simulink model "prelab10"  (R2021a)
settings: Solver=VariableStepAuto  StartTime=0.0  StopTime=0.005  RelTol=1e-3
settings Model: Creator=Mataya  LastModifiedBy=Mataya

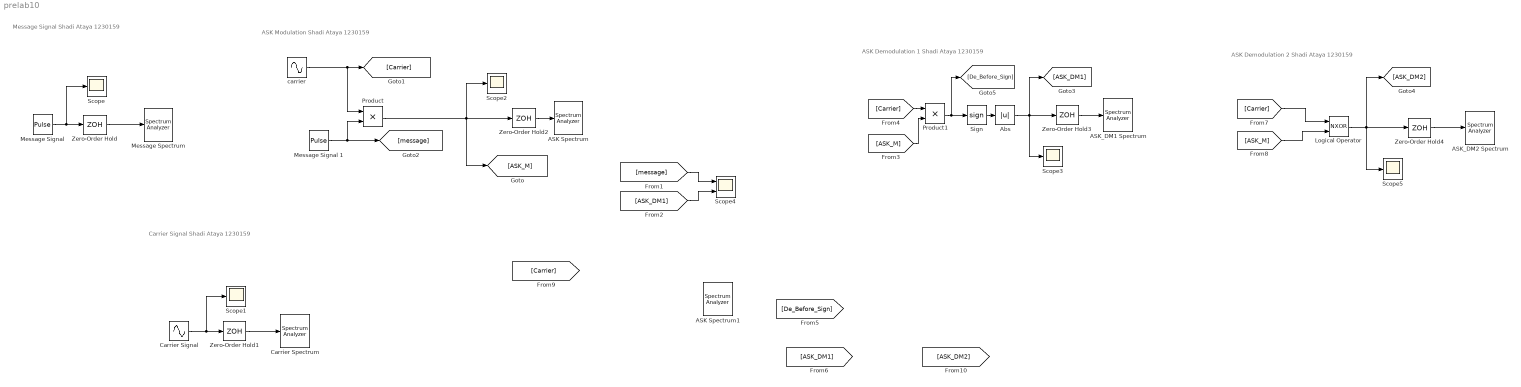
== system prelab10 ==
  note: ASK Demodulation 2
      | Shadi Ataya 1230159
  note: ASK Demodulation 1
      | Shadi Ataya 1230159
  note: ASK Modulation
      | Shadi Ataya 1230159
  note: Message Signal
      | Shadi Ataya 1230159
  note: Carrier Signal
      | Shadi Ataya 1230159
  ASK Spectrum : SpectrumAnalyzer
  ASK Spectrum1 : SpectrumAnalyzer
  ASK_DM1 Spectrum : SpectrumAnalyzer
  ASK_DM2 Spectrum : SpectrumAnalyzer
  Abs : Abs
  Carrier Spectrum : SpectrumAnalyzer
  Carrier Signal : Sin  Frequency=20000*2*pi  Phase=pi/2  SampleTime=0
  Logical Operator : Logic  Operator=NXOR  AllPortsSameDT=off  OutDataTypeStr=boolean
  Message Spectrum : SpectrumAnalyzer
  "Message Signal " : DiscretePulseGenerator  PulseType=Time based  Amplitude=5  Period=0.001  PulseWidth=50
  Message Signal 1 : DiscretePulseGenerator  PulseType=Time based  Amplitude=5  Period=0.001  PulseWidth=50
  Product : Product
  Product1 : Product
  Scope{,1..3,5} (5 alike) : Scope
  Scope4 : Scope  NumInputPorts=2
  Sign : Signum
  Zero-Order Hold : ZeroOrderHold  SampleTime=1/40000
  Zero-Order Hold{1..4} (4 alike) : ZeroOrderHold  SampleTime=1/60000
  "carrier " : Sin  Frequency=2*pi*20000  Phase=pi/2  SampleTime=0
  wires:
  "Message Signal "/1 -> Zero-Order Hold/1, Scope/1
  Zero-Order Hold/1 -> Message Spectrum/1
  Zero-Order Hold1/1 -> Carrier Spectrum/1
  Carrier Signal/1 -> Scope1/1, Zero-Order Hold1/1
  "carrier "/1 -> Product/1, [Carrier]
  Product/1 -> [ASK_M], Scope2/1, Zero-Order Hold2/1
  Zero-Order Hold2/1 -> ASK Spectrum/1
  Message Signal 1/1 -> [message], Product/2
  Product1/1 -> [De_Before_Sign], Sign/1
  [ASK_M] -> Product1/2
  Zero-Order Hold3/1 -> ASK_DM1 Spectrum/1
  Abs/1 -> Scope3/1, Zero-Order Hold3/1, [ASK_DM1]
  [Carrier] -> Product1/1
  Sign/1 -> Abs/1
  [message] -> Scope4/1
  [ASK_DM1] -> Scope4/2
  Zero-Order Hold4/1 -> ASK_DM2 Spectrum/1
  [ASK_M] -> Logical Operator/2
  [Carrier] -> Logical Operator/1
  Logical Operator/1 -> Zero-Order Hold4/1, [ASK_DM2], Scope5/1
